simulink model "SMTorqueControl_PdM"  (R2026a)
settings: Solver=FixedStepDiscrete  StopTime=1  FixedStep=Ts  EnableMultiTasking=on
PreLoadFcn:
  | if exist(fullfile(pwd, 'Ortak_Veri_ve_Parametreler'), 'dir'), addpath(fullfile(pwd, 'Ortak_Veri_ve_Parametreler')); end
  | if exist(fullfile(pwd, '..', 'Ortak_Veri_ve_Parametreler'), 'dir'), addpath(fullfile(pwd, '..', 'Ortak_Veri_ve_Parametreler')); end
  | if exist(fullfile(pwd, 'Mat_Dosyalari'), 'dir'), addpath(fullfile(pwd, 'Mat_Dosyalari')); end
  | SMTorqueControlData;
  | if ~exist('Cdc_PdM','var'), Cdc_PdM = Cdc; end;
  | if ~exist('ESR_PdM','var'), ESR_PdM = 1e-4; end;
  | if ~exist('Rbat_PdM','var'), Rbat_PdM = 1e-3; end;
  | if ~exist('Rs_PdM','var'), Rs_PdM = Rs; end;
  | if ~exist('Lad_PdM','var'), Lad_PdM = Lad; end;
  | if ~exist('Rfd_PdM','var'), Rfd_PdM = Rfd; end;
  | if ~exist('Gate_Fault_Mask','var'), Gate_Fault_Mask = [1;1;1;1;1;1]; end;
  | if ~exist('Stator_Unbalance_Gain','var'), Stator_Unbalance_Gain = [1;1;1]; end;
  | if ~exist('Load_Scale_PdM','var'), Load_Scale_PdM = 1.0; end;
  | if ~exist('Sensor_Offset_Drift_PdM','var'), Sensor_Offset_Drift_PdM = [0;0;0]; end;
InitFcn:
  | if exist(fullfile(pwd, 'Ortak_Veri_ve_Parametreler'), 'dir'), addpath(fullfile(pwd, 'Ortak_Veri_ve_Parametreler')); end
  | if exist(fullfile(pwd, '..', 'Ortak_Veri_ve_Parametreler'), 'dir'), addpath(fullfile(pwd, '..', 'Ortak_Veri_ve_Parametreler')); end
  | if exist(fullfile(pwd, 'Mat_Dosyalari'), 'dir'), addpath(fullfile(pwd, 'Mat_Dosyalari')); end
  | SMTorqueControlData;
  | if ~exist('Cdc_PdM','var'), Cdc_PdM = Cdc; end;
  | if ~exist('ESR_PdM','var'), ESR_PdM = 1e-4; end;
  | if ~exist('Rbat_PdM','var'), Rbat_PdM = 1e-3; end;
  | if ~exist('Rs_PdM','var'), Rs_PdM = Rs; end;
  | if ~exist('Lad_PdM','var'), Lad_PdM = Lad; end;
  | if ~exist('Rfd_PdM','var'), Rfd_PdM = Rfd; end;
  | if ~exist('Gate_Fault_Mask','var'), Gate_Fault_Mask = [1;1;1;1;1;1]; end;
  | if ~exist('Stator_Unbalance_Gain','var'), Stator_Unbalance_Gain = [1;1;1]; end;
  | if ~exist('Load_Scale_PdM','var'), Load_Scale_PdM = 1.0; end;
  | if ~exist('Sensor_Offset_Drift_PdM','var'), Sensor_Offset_Drift_PdM = [0;0;0]; end;
undefined symbols (not defined in the file): denZC_id, denZC_if, denZC_iq, ee_sli_rtmsupport, fsw, gcbh, Ibase, ID_MAP, IF_MAP, Ifbase, IQ_MAP, Kaw_id, Kaw_if, Kaw_iq, Ki_id, Ki_if, Ki_iq, Kp_id, Kp_if, Kp_iq, L_base, Lad, Ld, Lq, numZC_id, numZC_if, numZC_iq, p, Pmax, RPM_VECT, Tbase, TQ_VECT, Ts, Tsi, VDC_VECT, Vnom
libraries: nesl_utility x16, fl_lib x11, ee_lib x6, eeGeneralControl x3, eeTransforms x2, deeplib x2, sl_discontinuities x2, SignalEditorBlockLib x2, eeDqVoltageLimiter x1, simulink x1, sl_signal_attributes x1, eePwmGenerator x1
(part 1 of 2)
Description:
  | SM Torque Control
settings Model: Creator=The MathWorks, Inc.  LastModifiedBy=Dogukan.kilinc
settings DataIOCC: MaxDataPoints=210000  SignalLoggingName=logsout_SMTorqueControl
settings SimscapeCC: SimscapeNominalValues="[{\"value\":\"1\",\"unit\":\"A\"},{\"value\":\"1\",\"unit\":\"bar\"},{\"value\":\"1\",\"unit\":\"cm^2\"},{\"value\":\"1\",\"unit\":\"cm^3/s\"},{\"value\":\"1\",\"unit\":\"kJ/kg\"},{\"value\":\"1\",\"unit\":\"kW\"},{\"value\":\"1\",\"unit\":\"l\"},{\"value\":\"1\",\"unit\":\"N\"},{\"value\":\"1\",\"unit\":\"N*m\"},{\"value\":\"1\",\"unit\":\"V\"}]"  SimscapeLogType=none  SimscapeLogSimulationStatistics=on  SimscapeLogName=simlog_SMTorqueControl  SimscapeLogDataHistory=210000.0

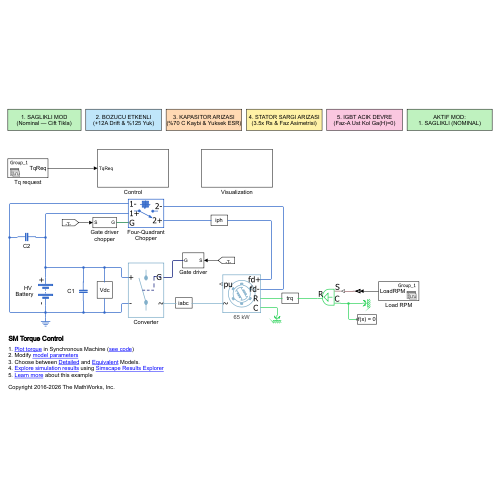
[thumbnail: Simulink's stored preview of the top-level diagram]
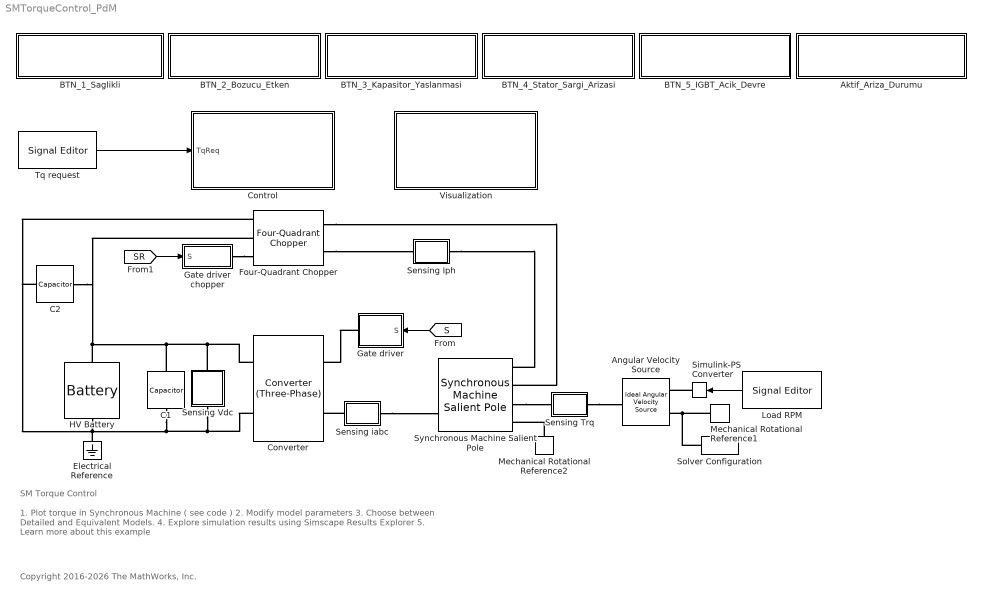
== system SMTorqueControl_PdM ==
  note: SM Torque Control
  note: 1. Plot torque in Synchronous Machine ( see code )
      | 2. Modify model parameters
      | 3. Choose between Detailed and Equivalent Models.
      | 4. Explore simulation results using Simscape Results Explorer
      | 5. Learn more about this example
  note: Copyright 2016-2026 The MathWorks, Inc.
  Aktif_Ariza_Durumu : Subsystem
      settings: OpenFcn=fprintf('[SMTorqueControl_PdM] Soldaki 5 renkli butondan birine cift tiklayarak ariza modunu degistirebilirsiniz.\\n');
      mask Display: disp(['AKTIF MOD:' newline '1. SAGLIKLI (NOMINAL)'])
  Angular Velocity Source : fl_lib/Mechanical/Mechanical Sources/Ideal Angular Velocity Source
  BTN_1_Saglikli : Subsystem
      settings: OpenFcn=|
      | evalin('base', 'if ~exist(''Cdc'',''var''), SMTorqueControlData; end;');
      | evalin('base', 'Cdc_PdM=Cdc; ESR_PdM=1e-3; Rbat_PdM=1e-3; Rs_PdM=Rs; Lad_PdM=Lad; Rfd_PdM=Rfd; Gate_Fault_Mask=[1;1;1;1;1;1]; Stator_Unbalance_Gain=[1;1;1]; Sensor_Offset_Drift_PdM=[0;0;0]; Load_Scale_PdM=1.0;');
      | set_param('SMTorqueControl_PdM/Gate driver/IGBT_Kanal_Maskesi', 'Value', '[1;1;1;1;1;1]');
      | set_param('SMTorqueControl_PdM/Control/Measurements/Stator_Faz_Asimetri_Enjektoru', 'Gain', '[1;1;1]');
      | set_param('SMTorqueControl_PdM/Control/Measurements/Sensor_Bozucu_Ofset', 'Value', '[0;0;0]');
      | set_param('SMTorqueControl_PdM/Control/Yuk_Olcekleyici', 'Gain', '1.0');
      | set_param('SMTorqueControl_PdM/Aktif_Ariza_Durumu', 'MaskDisplay', 'disp([''AKTIF MOD:'' newline ''1. SAGLIKLI (NOMINAL)''])', 'BackgroundColor', '[0.75 0.95 0.75]');
      | if strcmp(get_param('SMTorqueControl_PdM','SimulationStatus'),'running'), set_param('SMTorqueControl_PdM','SimulationCommand','update'); end;
      | fprintf('[SMTorqueControl_PdM] >>> Mod 1 Secildi: SAGLIKLI (NOMINAL) MOD aktif!\n');
      mask Display: disp('1. SAGLIKLI MOD\n(Nominal — Cift Tikla)')
  BTN_2_Bozucu_Etken : Subsystem
      settings: OpenFcn=|
      | evalin('base', 'if ~exist(''Cdc'',''var''), SMTorqueControlData; end;');
      | evalin('base', 'Cdc_PdM=Cdc; ESR_PdM=1e-3; Rbat_PdM=1e-3; Rs_PdM=Rs; Lad_PdM=Lad; Rfd_PdM=Rfd; Gate_Fault_Mask=[1;1;1;1;1;1]; Stator_Unbalance_Gain=[1.04;0.98;0.98]; Sensor_Offset_Drift_PdM=[12;-6;-6]; Load_Scale_PdM=1.25;');
      | set_param('SMTorqueControl_PdM/Gate driver/IGBT_Kanal_Maskesi', 'Value', '[1;1;1;1;1;1]');
      | set_param('SMTorqueControl_PdM/Control/Measurements/Stator_Faz_Asimetri_Enjektoru', 'Gain', '[1.04;0.98;0.98]');
      | set_param('SMTorqueControl_PdM/Control/Measurements/Sensor_Bozucu_Ofset', 'Value', '[12;-6;-6]');
      | set_param('SMTorqueControl_PdM/Control/Yuk_Olcekleyici', 'Gain', '1.25');
      | set_param('SMTorqueControl_PdM/Aktif_Ariza_Durumu', 'MaskDisplay', 'disp([''AKTIF MOD:'' newline ''2. BOZUCU ETKEN (+12A, %125)''])', 'BackgroundColor', '[0.75 0.90 0.98]');
      | if strcmp(get_param('SMTorqueControl_PdM','SimulationStatus'),'running'), set_param('SMTorqueControl_PdM','SimulationCommand','update'); end;
      | fprintf('[SMTorqueControl_PdM] >>> Mod 2 Secildi: BOZUCU ETKENLI SAGLIKLI MOD (+12A Drift, %%125 Yuk) aktif!\n');
      mask Display: disp('2. BOZUCU ETKENLI\n(+12A Drift & %125 Yuk)')
  BTN_3_Kapasitor_Yaslanmasi : Subsystem
      settings: OpenFcn=|
      | evalin('base', 'if ~exist(''Cdc'',''var''), SMTorqueControlData; end;');
      | evalin('base', 'Cdc_PdM=0.30*Cdc; ESR_PdM=0.08; Rbat_PdM=0.18; Rs_PdM=Rs; Lad_PdM=Lad; Rfd_PdM=Rfd; Gate_Fault_Mask=[1;1;1;1;1;1]; Stator_Unbalance_Gain=[1;1;1]; Sensor_Offset_Drift_PdM=[0;0;0]; Load_Scale_PdM=1.0;');
      | set_param('SMTorqueControl_PdM/Gate driver/IGBT_Kanal_Maskesi', 'Value', '[1;1;1;1;1;1]');
      | set_param('SMTorqueControl_PdM/Control/Measurements/Stator_Faz_Asimetri_Enjektoru', 'Gain', '[1;1;1]');
      | set_param('SMTorqueControl_PdM/Control/Measurements/Sensor_Bozucu_Ofset', 'Value', '[0;0;0]');
      | set_param('SMTorqueControl_PdM/Control/Yuk_Olcekleyici', 'Gain', '1.0');
      | set_param('SMTorqueControl_PdM/Aktif_Ariza_Durumu', 'MaskDisplay', 'disp([''AKTIF MOD:'' newline ''3. KAPASITOR YASLANMASI''])', 'BackgroundColor', '[1.00 0.85 0.70]');
      | if strcmp(get_param('SMTorqueControl_PdM','SimulationStatus'),'running'), set_param('SMTorqueControl_PdM','SimulationCommand','update'); end;
      | fprintf('[SMTorqueControl_PdM] >>> Mod 3 Secildi: DC-LINK KAPASITOR YASLANMASI aktif!\n');
      mask Display: disp('3. KAPASITOR ARIZASI\n(%70 C Kaybi & Yuksek ESR)')
  BTN_4_Stator_Sargi_Arizasi : Subsystem
      settings: OpenFcn=|
      | evalin('base', 'if ~exist(''Cdc'',''var''), SMTorqueControlData; end;');
      | evalin('base', 'Cdc_PdM=Cdc; ESR_PdM=1e-3; Rbat_PdM=1e-3; Rs_PdM=3.5*Rs; Lad_PdM=0.82*Lad; Rfd_PdM=1.4*Rfd; Gate_Fault_Mask=[1;1;1;1;1;1]; Stator_Unbalance_Gain=[1.12;0.94;0.94]; Sensor_Offset_Drift_PdM=[0;0;0]; Load_Scale_PdM=1.0;');
      | set_param('SMTorqueControl_PdM/Gate driver/IGBT_Kanal_Maskesi', 'Value', '[1;1;1;1;1;1]');
      | set_param('SMTorqueControl_PdM/Control/Measurements/Stator_Faz_Asimetri_Enjektoru', 'Gain', '[1.12;0.94;0.94]');
      | set_param('SMTorqueControl_PdM/Control/Measurements/Sensor_Bozucu_Ofset', 'Value', '[0;0;0]');
      | set_param('SMTorqueControl_PdM/Control/Yuk_Olcekleyici', 'Gain', '1.0');
      | set_param('SMTorqueControl_PdM/Aktif_Ariza_Durumu', 'MaskDisplay', 'disp([''AKTIF MOD:'' newline ''4. STATOR SARGI ARIZASI''])', 'BackgroundColor', '[1.00 0.95 0.65]');
      | if strcmp(get_param('SMTorqueControl_PdM','SimulationStatus'),'running'), set_param('SMTorqueControl_PdM','SimulationCommand','update'); end;
      | fprintf('[SMTorqueControl_PdM] >>> Mod 4 Secildi: STATOR SARGI ARIZASI & FAZ ASIMETRISI aktif!\n');
      mask Display: disp('4. STATOR SARGI ARIZASI\n(3.5x Rs & Faz Asimetrisi)')
  BTN_5_IGBT_Acik_Devre : Subsystem
      settings: OpenFcn=|
      | evalin('base', 'if ~exist(''Cdc'',''var''), SMTorqueControlData; end;');
      | evalin('base', 'Cdc_PdM=Cdc; ESR_PdM=1e-3; Rbat_PdM=1e-3; Rs_PdM=Rs; Lad_PdM=Lad; Rfd_PdM=Rfd; Gate_Fault_Mask=[0;1;1;1;1;1]; Stator_Unbalance_Gain=[1;1;1]; Sensor_Offset_Drift_PdM=[0;0;0]; Load_Scale_PdM=1.0;');
      | set_param('SMTorqueControl_PdM/Gate driver/IGBT_Kanal_Maskesi', 'Value', '[0;1;1;1;1;1]');
      | set_param('SMTorqueControl_PdM/Control/Measurements/Stator_Faz_Asimetri_Enjektoru', 'Gain', '[1;1;1]');
      | set_param('SMTorqueControl_PdM/Control/Measurements/Sensor_Bozucu_Ofset', 'Value', '[0;0;0]');
      | set_param('SMTorqueControl_PdM/Control/Yuk_Olcekleyici', 'Gain', '1.0');
      | set_param('SMTorqueControl_PdM/Aktif_Ariza_Durumu', 'MaskDisplay', 'disp([''AKTIF MOD:'' newline ''5. INVERTER IGBT ARIZASI''])', 'BackgroundColor', '[0.98 0.78 0.88]');
      | if strcmp(get_param('SMTorqueControl_PdM','SimulationStatus'),'running'), set_param('SMTorqueControl_PdM','SimulationCommand','update'); end;
      | fprintf('[SMTorqueControl_PdM] >>> Mod 5 Secildi: INVERTER A-FAZI UST IGBT ACIK DEVRE ARIZASI aktif!\n');
      mask Display: disp('5. IGBT ACIK DEVRE\n(Faz-A Ust Kol Ga(H)=0)')
  C1 : fl_lib/Electrical/Electrical Elements/Capacitor  c=Cdc_PdM F  r=ESR_PdM Ohm  g=0 1/Ohm  i_specify=off  i_priority=None  i=0 A  i_nominal_specify=off  i_nominal_value=1  i_nominal_unit=A  v_specify=off  v_priority=None  v=0 V  v_nominal_specify=off  v_nominal_value=1  v_nominal_unit=V  vc_specify=on  vc_priority=None  vc=Vnom V  vc_nominal_specify=off  vc_nominal_value=1  vc_nominal_unit=V
  C2 : fl_lib/Electrical/Electrical Elements/Capacitor  c=Cdc_PdM F  r=ESR_PdM Ohm  g=0 1/Ohm  i_specify=off  i_priority=None  i=0 A  i_nominal_specify=off  i_nominal_value=1  i_nominal_unit=A  v_specify=off  v_priority=None  v=0 V  v_nominal_specify=off  v_nominal_value=1  v_nominal_unit=V  vc_specify=on  vc_priority=None  vc=Vnom V  vc_nominal_specify=off  vc_nominal_value=1  vc_nominal_unit=V
  Control : Subsystem
  Converter : ee_lib/Semiconductors & Converters/Converters/Converter (Three-Phase)  port_option=ee.enum.threePhasePort.composite  fidelity_option=ee.enum.converters.fidelity.detailed  device_type=2  showThermalPort=false  K=0  Vth=0.5 V  Vgt=1 V  Vgt_off=-1 V  Ih=1 A  Vf=0.8 V  Ron=0.001 Ohm  Rds=0.001 Ohm  Goff=1e-5 1/Ohm  Eon_scalar=22.86e-3 J  Eoff_scalar=17.14e-3 J  Eoff_natural_commutation=10e-3 J  Voff=300 V  Iout_scalar=600 A  onCurrentMeasDelay=0 s  useCurrentFromPreviousCycle=false  useVoltageFromPreviousCycle=false  diode_param=2  diode_Vf=0.8 V  diode_Ron=0.001 Ohm  diode_Goff=1e-5 1/Ohm  diode_C=50 nF  diode_iRM=-235 A  diode_iF=300 A  diode_idot=-50 A/us  diode_trr_param=1  diode_trr_factor=3  diode_trr=15 us  diode_Qrr=1.5e+3 s*uA  diode_rec_loss_model=ee.enum.diode.reverseRecoveryModel.fixed  diode_ErecVal=0 J  diode_scaleWithIandV=false  diode_ErecMat=zeros(2, 3) J  diode_TjrecVec=[298.15, 398.15] K  diode_IfrecVec=[.1, 1, 10] A  diode_IrecVal=10 A  diode_VrecVal=10 V  diode_tFilter=1 / 1000 / 100 s  thermal_network_parameterization=ee.enum.thermalNetworkTopology.external  Rth=[.08, .5] K/W  Rth_Cauer=[.08, .1, .5] K/W  Rth_Foster=[.08, .14, .22, .16] K/W  thermal_mass_parameterization=ee.enum.thermalNetwork.timeconstant  thermal_mass=[.01, .5] J/K  thermal_mass_Cauer=[.01, .1, .5] J/K  thermal_mass_Foster=[.001, .005, .05, .5] J/K  thermal_time_constant=[.001, .2] s  thermal_time_constant_Cauer=[.001, .1, .2] s  thermal_time_constant_Foster=[7e-05, .0007, .01, .08] s  thermal_mass_initial_temperatures=[25, 25] degC  thermal_mass_initial_temperatures_Cauer=[25, 25, 25] degC  junction_thermal_mass=0.01 J/K  Tvec_initial_Foster=[25, 25, 25, 25] degC  snubber_type=0  Cs=1e-7 F  Rs=0.1 Ohm  Vce_loss=[0, 150, 300] V
  Electrical Reference : fl_lib/Electrical/Electrical Elements/Electrical Reference
  Four-Quadrant Chopper : ee_lib/Semiconductors & Converters/Converters/Four-Quadrant Chopper  fidelity_option=ee.enum.converters.fidelity.detailed  device_type=3  showThermalPort=false  Vgt=1 V  Vgt_off=-1 V  Ih=1 A  Vf=0.8 V  Ron=0.001 Ohm  Rds=0.001 Ohm  Goff=1e-5 1/Ohm  Vth=0.5 V  K=0  Eon_scalar=22.86e-3 J  Eoff_scalar=17.14e-3 J  Eoff_natural_commutation=10e-3 J  Voff=300 V  Iout_scalar=600 A  onCurrentMeasDelay=0 s  useCurrentFromPreviousCycle=false  useVoltageFromPreviousCycle=false  diode_param=2  diode_Vf=0.8 V  diode_Ron=0.001 Ohm  diode_Goff=1e-5 1/Ohm  diode_C=50 nF  diode_iRM=-235 A  diode_iF=300 A  diode_idot=-50 A/us  diode_trr_param=1  diode_trr_factor=3  diode_trr=15 us  diode_Qrr=1500 s*uA  diode_rec_loss_model=ee.enum.diode.reverseRecoveryModel.fixed  diode_ErecVal=0 J  diode_scaleWithIandV=false  diode_ErecMat=zeros(2, 3) J  diode_TjrecVec=[298.15, 398.15] K  diode_IfrecVec=[.1, 1, 10] A  diode_IrecVal=10 A  diode_VrecVal=10 V  diode_tFilter=1 / 1000 / 100 s  thermal_network_parameterization=ee.enum.thermalNetworkTopology.external  Rth=[.08, .5] K/W  Rth_Cauer=[.08, .1, .5] K/W  Rth_Foster=[.08, .14, .22, .16] K/W  thermal_mass_parameterization=ee.enum.thermalNetwork.timeconstant  thermal_mass=[.01, .5] J/K  thermal_mass_Cauer=[.01, .1, .5] J/K  thermal_mass_Foster=[.001, .005, .05, .5] J/K  thermal_time_constant=[.001, .2] s  thermal_time_constant_Cauer=[.001, .1, .2] s  thermal_time_constant_Foster=[7e-05, .0007, .01, .08] s  thermal_mass_initial_temperatures=[25, 25] degC  thermal_mass_initial_temperatures_Cauer=[25, 25, 25] degC  junction_thermal_mass=0.01 J/K  Tvec_initial_Foster=[25, 25, 25, 25] degC  snubber_type=0  Cs=1e-7 F  Rs=0.1 Ohm
  Gate driver : Subsystem
  Gate driver chopper : Subsystem
  HV Battery : batteryecm_lib/Battery  Vnom=Vnom V  prm_dir=1  R1_dis=2 Ohm  R1_ch=2 Ohm  R1=Rbat_PdM Ohm  prm_AH=1  AH=300 hr*A  V1=330 V  AH1=100 hr*A  prm_R2=1  R2=2000 Ohm  Tmeas=298.15 K  charge_measurement_port=simscape.enum.battery.enable.no  prm_dyn=1  Rp1=0.005 Ohm  tau1=30 s  Rp2=0.005 Ohm  tau2=30 s  Rp3=0.005 Ohm  tau3=30 s  Rp4=0.005 Ohm  tau4=30 s  Rp5=0.005 Ohm  tau5=30 s  prm_fade=1  N_fade=100  AH_fade=45 hr*A  R1_fade=2.02 Ohm  R1_ch_fade=2.02 Ohm  V1_fade=10.35 V  prm_age=1  prm_age_OCV=1  OCV_age=0.9  SOC_age=60  Tmeas_age=298.15 K  delta_time_age_vec=[0] d  temperature_age_vec=[273] K  OCV_scaling_age=2.2134e6  OCV_offset_age=1.632e6  temp_exp_age=0.515833569 V  t_exp_age=0.75  Vnom_T2=12 V  R1_T2=2.2 Ohm  R1_T2_dis=2.2 Ohm  R1_T2_ch=2.2 Ohm  V1_T2=11.4 V  R2_T2=2200 Ohm  Rp1_T2=0.005 Ohm  tau1_T2=30 s  Rp2_T2=0.005 Ohm  tau2_T2=30 s  Rp3_T2=0.005 Ohm  tau3_T2=30 s  Rp4_T2=0.005 Ohm  tau4_T2=30 s  Rp5_T2=0.005 Ohm  tau5_T2=30 s  Tmeas2=273.15 K  thermal_port=simscape.enum.thermaleffects.omit  thermal_mass=30000 J/K  i_specify=off  i_priority=None  i=0 A  i_nominal_specify=off  i_nominal_value=1  i_nominal_unit=A  v_specify=off  v_priority=None  v=0 V  v_nominal_specify=off  v_nominal_value=1  v_nominal_unit=V  charge_specify=on  charge_priority=High  charge=AH0 hr*A  charge_nominal_specify=off  charge_nominal_value=1  charge_nominal_unit=A*hr  num_cycles_specify=off  num_cycles_priority=High  num_cycles=0  num_cycles_nominal_specify=off  num_cycles_nominal_value=1  num_cycles_nominal_unit=1  temperature_specify=off  temperature_priority=High  temperature=298.15 K  temperature_nominal_specify=off  temperature_nominal_value=1  temperature_nominal_unit=K
  Load RPM : SignalEditorBlockLib/Signal Editor  FileName=SMTorqueControlLoadRPM.mat  ActiveScenario=Group_1  ActiveSignal=LoadRPM  IsBus=off  OutputBusObjectStr=Bus: BusObject  SampleTime=0  OutputAfterFinalValue=Extrapolation  Unit=inherit  PreserveSignalName=on  ApplySigPropsToAllScenarios=on  ApplySigPropsToAllSignals=off  SignalPropertySource=Dialog parameters
  Mechanical Rotational Reference1 : fl_lib/Mechanical/Rotational Elements/Mechanical Rotational Reference
  Mechanical Rotational Reference2 : fl_lib/Mechanical/Rotational Elements/Mechanical Rotational Reference
  Sensing Iph : Subsystem
      mask Display: disp('iph')
  Sensing Trq : Subsystem
      mask Display: disp('trq')
  Sensing Vdc : Subsystem
      mask Display: disp('Vdc')
  Sensing iabc : Subsystem
      mask Display: disp('iabc')
  Simulink-PS Converter : nesl_utility/Simulink-PS Converter  PhysicalDomain=network_engine_domain  SubClassName=ps_input  LeftPortType=input  RightPortType=output  PseudoPeriodic=off  Frequencies=[]  NoiseDistribution=none  NoiseParameters=[]  Unit=rpm  AffineConversion=off  FilteringAndDerivatives=zero  SimscapeFilterOrder=1  InputFilterTimeConstant=0.001  UdotUserProvided=1
  Solver Configuration : nesl_utility/Solver Configuration  PhysicalDomain=network_engine_domain  SubClassName=solver  LeftPortType=input  RightPortType=generic  Tones=[]  Harmonics=[]  SimulateNoise=off  Profile=off  UseLocalSampling=off  EnableSwitchedLinearOptims=on  FrequencyDomain=off  UseCCode=off  RelTol=0.001  AbsTol=1e-06  MinStep=1e-09  ToWorkspace=off  RevertToSquareIcSolve=off  NumHomotopyIterations=100  PhasorMode=off  PhasorModeNumHarmonics=1  ConsistencySolver=NEWTON_FTOL  CanonicalOrdering=UNORDERED  OptimizeIntermediates=UNOPTIMIZED  IndexReductionMethod=DerivativeReplacement  DoDC=off  ResidualTolerance=1e-9  ConsistencyTolSource=GLOBAL  ConsistencyAbsTol=0.001  ConsistencyRelTol=0.001  ConsistencyTolFactor=0.001  UseLocalSolver=on  LocalSolverChoice=NE_BACKWARD_EULER_ADVANCER  ResolveIndetEquations=on  FunctionEvalNumThread=1  LocalSolverSampleTime=Ts  DoFixedCost=on  MaxNonlinIter=4  MaxModeIter=2  ComputeImpulses=off  ImpulseIterations=2  LinearAlgebra=auto  LinearAlgebraNumThread=0  EquationFormulation=NE_TIME_EF  DelaysMemoryBudget=1024  AutomaticFiltering=on  FilteringTimeConstant=0.001  PartitionStorageMethod=AS_NEEDED  PartitionMemoryBudget=1024  PartitionMethod=FAST  MultibodyUseLocalSolver=off  MultibodyLocalSolverChoice=ODE1  MultibodyLocalSolverSampleTime=0.001
  Synchronous Machine Salient Pole : ee_lib/Electromechanical/Synchronous/Synchronous Machine Salient Pole  port_option=ee.enum.threePhasePort.composite  SRated=Pmax W  VRated=Vr V  FRated=fr Hz  nPolePairs=p  param_option=ee.enum.sm.parameterization.fundamental  fieldCircuitParameterization_option=2  baseEfd=272 V  baseIfd=Ifbase A  zero_sequence=ee.enum.park.zerosequence.exclude  axes_param=ee.enum.rotorangle.daxis  Ladu=Lad_PdM  Laqu=Laq  L0=L0  Ll=Ll  Ra=Rs_PdM  Lfd=Lfd  Rfd=Rfd_PdM  L1d=0.1  R1d=0.254  L1q=0.1567  R1q=0.328  Xl=0.15  Xd=1.05  Xq=0.7  X0=0.15  Xdd=0.35  Xddd=0.25  Xqdd=0.325  d_option=ee.enum.circuit.open  Td0d=5.25 s  Tdd=1.75 s  Td0dd=0.03 s  Tddd=0.0214 s  q_option=ee.enum.circuit.open  Tq0dd=0.05 s  Tqdd=0.0232 s  saturation_option=0  saturation_ifd=[0.0, 0.48, 0.76, 1.38, 1.79]  saturation_Vag=[0.0, 0.43, 0.59, 0.71, 0.76]  initialization_option=1  source_type=ee.enum.sm.load_flow_source_type.Swing  Vmag0=Vr V  Vang0=0 deg  Pt0=0 V*A  Qt0=0 V*A  minimum_pu=0.95  phase_search_range=[-30, 30] deg  gmin=1e-6 S  connection_option=ee.enum.Connection.wye  num_q_dampers=1  rotor_offset=-pi / 2 rad  pu_psid_specify=on  pu_psid_priority=High  pu_psid=0  pu_psid_nominal_specify=off  pu_psid_nominal_value=1  pu_psid_nominal_unit=1  pu_psiq_specify=on  pu_psiq_priority=High  pu_psiq=0  pu_psiq_nominal_specify=off  pu_psiq_nominal_value=1  pu_psiq_nominal_unit=1  pu_psifd_specify=on  pu_psifd_priority=High  pu_psifd=0  pu_psifd_nominal_specify=off  pu_psifd_nominal_value=1  pu_psifd_nominal_unit=1  pu_psi1d_specify=on  pu_psi1d_priority=High  pu_psi1d=0  pu_psi1d_nominal_specify=off  pu_psi1d_nominal_value=1  pu_psi1d_nominal_unit=1  pu_psi1q_specify=on  pu_psi1q_priority=High  pu_psi1q=0  pu_psi1q_nominal_specify=off  pu_psi1q_nominal_value=1  pu_psi1q_nominal_unit=1  angular_position_diff_specify=on  angular_position_diff_priority=High  angular_position_diff=-pi/2/p rad  angular_position_diff_nominal_specify=off  angular_position_diff_nominal_value=1  angular_position_diff_nominal_unit=deg  Tmeas=298.15 K  alpha=3.93e-3 1/K  stator_thermal_mass=100 J/K  rotor_thermal_mass=200 J/K  temperatureA_specify=off  temperatureA_priority=High  temperatureA=25 degC  temperatureA_nominal_specify=off  temperatureA_nominal_value=1  temperatureA_nominal_unit=degC  temperatureB_specify=off  temperatureB_priority=High  temperatureB=25 degC  temperatureB_nominal_specify=off  temperatureB_nominal_value=1  temperatureB_nominal_unit=degC  temperatureC_specify=off  temperatureC_priority=High  temperatureC=25 degC  temperatureC_nominal_specify=off  temperatureC_nominal_value=1  temperatureC_nominal_unit=degC  temperatureR_specify=off  temperatureR_priority=High  temperatureR=25 degC  temperatureR_nominal_specify=off  temperatureR_nominal_value=1  temperatureR_nominal_unit=degC
      settings: AttributesFormatString=65 kW
  Tq request : SignalEditorBlockLib/Signal Editor  FileName=SMTorqueControlTorqueRequest.mat  ActiveScenario=Group_1  ActiveSignal=TqReq  IsBus=off  OutputBusObjectStr=Bus: BusObject  SampleTime=0  OutputAfterFinalValue=Extrapolation  Unit=inherit  PreserveSignalName=on  ApplySigPropsToAllScenarios=on  ApplySigPropsToAllSignals=off  SignalPropertySource=Dialog parameters
  Visualization : Subsystem
  wires:
  [S] -> Gate driver/1(S)
  Load RPM/1 -> Simulink-PS Converter/1
  [SR] -> Gate driver chopper/1(S)
  Tq request/1 -> Control/1(TqReq)
  connections:
  Sensing Trq/RConn1 -- Angular Velocity Source/LConn1
  Converter/RConn2 -- Sensing Vdc/RConn1 -- Four-Quadrant Chopper/LConn3 -- C2/RConn1 -- HV Battery/RConn1 -- Electrical Reference/LConn1 -- C1/RConn1
  Converter/RConn1 -- Sensing Vdc/LConn1 -- Four-Quadrant Chopper/LConn2 -- C2/LConn1 -- HV Battery/LConn1 -- C1/LConn1
  Gate driver/RConn1 -- Converter/LConn1
  Simulink-PS Converter/RConn1 -- Angular Velocity Source/RConn1
  Synchronous Machine Salient Pole/LConn3 -- Sensing Trq/LConn1
  Mechanical Rotational Reference1/LConn1 -- Solver Configuration/RConn1 -- Angular Velocity Source/RConn2
  Four-Quadrant Chopper/RConn1 -- Sensing Iph/LConn1
  Four-Quadrant Chopper/RConn2 -- Synchronous Machine Salient Pole/LConn2
  Sensing Iph/RConn1 -- Synchronous Machine Salient Pole/LConn1
  Sensing iabc/LConn1 -- Converter/LConn2
  Sensing iabc/RConn1 -- Synchronous Machine Salient Pole/RConn2
  Gate driver chopper/RConn1 -- Four-Quadrant Chopper/LConn1
  Mechanical Rotational Reference2/LConn1 -- Synchronous Machine Salient Pole/LConn4

== system SMTorqueControl_PdM/Aktif_Ariza_Durumu ==

== system SMTorqueControl_PdM/BTN_1_Saglikli ==

== system SMTorqueControl_PdM/BTN_2_Bozucu_Etken ==

== system SMTorqueControl_PdM/BTN_3_Kapasitor_Yaslanmasi ==

== system SMTorqueControl_PdM/BTN_4_Stator_Sargi_Arizasi ==

== system SMTorqueControl_PdM/BTN_5_IGBT_Acik_Devre ==

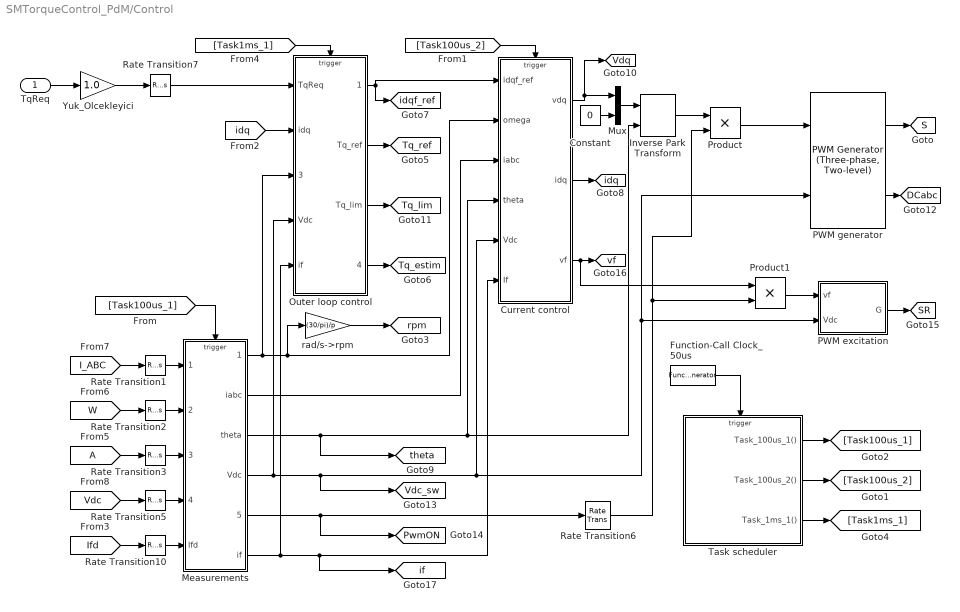
== system SMTorqueControl_PdM/Control ==
  TqReq : Inport
  Constant : Constant  Value=0  SampleTime=-1
  Current control : Subsystem
  From5 : From  TagVisibility=global
  Function-Call Clock_50us : FunctionCallGenerator  SampleTime=5e-5
  Inverse Park Transform : eeTransforms/Inverse Park Transform  AxisAlignment=Q-axis  PowerInvariant=off
  Measurements : Subsystem
  Mux : Mux  Inputs=2
  Outer loop control : Subsystem
  PWM excitation : Subsystem
  PWM generator : eePwmGeneratorTwoLevel/PWM Generator (Three-phase, Two-level)  PWMMode=Continuous PWM (CPWM)  CPWMMode=SVM: space vector modulation  DPWMMode=60 DPWM: 60 degree discontinuous PWM  fsw=fsw  Ts=Ts
  Product : Product
  Product1 : Product
  Rate Transition{1..3,5..7,10} (7 alike) : RateTransition
  Task scheduler : Stateflow chart  TreatAsAtomicUnit=on
  Yuk_Olcekleyici : Gain  Gain=1.0
  rad/s->rpm : Gain  Gain=(30/pi)/p
  tag scope: DCabc=global, PwmON=global, S=global, SR=global, Tq_estim=global, Tq_lim=global, Tq_ref=global, Vdc_sw=global, Vdq=global, idq=global, idqf_ref=global, if=global, rpm=global, theta=global, vf=global
  wires:
  [Ifd] -> Rate Transition10/1
  [W] -> Rate Transition2/1
  [idq] -> Outer loop control/2(idq)
  [Task100us_1] -> Measurements/Trigger
  Measurements/5(PwmON) -> Rate Transition6/1, [PwmON]
  Rate Transition1/1 -> Measurements/1(iabc_m)
  PWM generator/2 -> [DCabc]
  [I_ABC] -> Rate Transition1/1
  Rate Transition6/1 -> Product1/2, Product/2
  [Task100us_2] -> Current control/Trigger
  Measurements/2(iabc) -> Current control/3(iabc)
  Outer loop control/4(Tq_estim) -> [Tq_estim]
  Current control/3(vf) -> Product1/1, [vf]
  Measurements/1(omega) -> rad/s->rpm/1, Current control/2(omega), Outer loop control/3(omega)
  rad/s->rpm/1 -> [rpm]
  Current control/2(idq) -> [idq]
  Rate Transition10/1 -> Measurements/5(Ifd)
  Task scheduler/2(Task_100us_2()) -> [Task100us_2]
  From5/1 -> Rate Transition3/1
  Measurements/3(theta) -> [theta], Inverse Park Transform/2, Current control/4(theta)
  Outer loop control/2(Tq_ref) -> [Tq_ref]
  Task scheduler/1(Task_100us_1()) -> [Task100us_1]
  [Task1ms_1] -> Outer loop control/Trigger
  Rate Transition2/1 -> Measurements/2(omega_m)
  Task scheduler/3(Task_1ms_1()) -> [Task1ms_1]
  Measurements/4(Vdc) -> [Vdc_sw], PWM generator/2, PWM excitation/2(Vdc), Current control/5(Vdc), Outer loop control/4(Vdc)
  [Vdc] -> Rate Transition5/1
  Rate Transition5/1 -> Measurements/4(Vdc_m)
  PWM generator/1 -> [S]
  Rate Transition3/1 -> Measurements/3(theta_m)
  Outer loop control/3(Tq_lim) -> [Tq_lim]
  Measurements/6(if) -> [if], Current control/6(If), Outer loop control/5(if)
  PWM excitation/1(G) -> [SR]
  Function-Call Clock_50us/1 -> Task scheduler/Trigger
  Outer loop control/1(idqf_ref) -> Current control/1(idqf_ref), [idqf_ref]
  Constant/1 -> Mux/2
  Mux/1 -> Inverse Park Transform/1
  Current control/1(vdq) -> [Vdq], Mux/1
  Product/1 -> PWM generator/1
  Inverse Park Transform/1 -> Product/1
  Product1/1 -> PWM excitation/1(vf)
  TqReq/1 -> Yuk_Olcekleyici/1
  Yuk_Olcekleyici/1 -> Rate Transition7/1
  Rate Transition7/1 -> Outer loop control/1(TqReq)

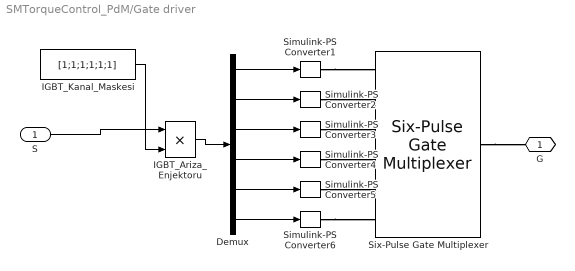
== system SMTorqueControl_PdM/Gate driver ==
  S : Inport
  Demux : Demux  Outputs=6
  IGBT_Ariza_Enjektoru : Product  Inputs=**
  IGBT_Kanal_Maskesi : Constant  Value=[1;1;1;1;1;1]
  Simulink-PS Converter{1..6} (6 alike) : nesl_utility/Simulink-PS Converter  PhysicalDomain=network_engine_domain  SubClassName=ps_input  LeftPortType=input  RightPortType=output  PseudoPeriodic=off  Frequencies=[]  NoiseDistribution=none  NoiseParameters=[]  Unit=1  AffineConversion=off  FilteringAndDerivatives=zero  SimscapeFilterOrder=1  InputFilterTimeConstant=0.001  UdotUserProvided=1
  Six-Pulse Gate Multiplexer : ee_lib/Semiconductors & Converters/Converters/Six-Pulse Gate Multiplexer  port_option=ee.enum.controlport.ps
  G : PMIOPort  Side=Right
  wires:
  Demux/1 -> Simulink-PS Converter1/1
  Demux/4 -> Simulink-PS Converter4/1
  Demux/2 -> Simulink-PS Converter2/1
  Demux/3 -> Simulink-PS Converter3/1
  Demux/5 -> Simulink-PS Converter5/1
  Demux/6 -> Simulink-PS Converter6/1
  S/1 -> IGBT_Ariza_Enjektoru/1
  IGBT_Kanal_Maskesi/1 -> IGBT_Ariza_Enjektoru/2
  IGBT_Ariza_Enjektoru/1 -> Demux/1
  connections:
  Six-Pulse Gate Multiplexer/RConn1 -- G/RConn1
  Simulink-PS Converter1/RConn1 -- Six-Pulse Gate Multiplexer/LConn1
  Simulink-PS Converter3/RConn1 -- Six-Pulse Gate Multiplexer/LConn3
  Simulink-PS Converter5/RConn1 -- Six-Pulse Gate Multiplexer/LConn5
  Simulink-PS Converter6/RConn1 -- Six-Pulse Gate Multiplexer/LConn6
  Simulink-PS Converter4/RConn1 -- Six-Pulse Gate Multiplexer/LConn4
  Simulink-PS Converter2/RConn1 -- Six-Pulse Gate Multiplexer/LConn2

== system SMTorqueControl_PdM/Gate driver chopper ==
  S : Inport
  Demux : Demux  Outputs=2
  Four-Pulse Gate Multiplexer : ee_lib/Semiconductors & Converters/Converters/Four-Pulse Gate Multiplexer  port_option=ee.enum.controlport.ps
  Simulink-PS Converter1 : nesl_utility/Simulink-PS Converter  PhysicalDomain=network_engine_domain  SubClassName=ps_input  LeftPortType=input  RightPortType=output  PseudoPeriodic=off  Frequencies=[]  NoiseDistribution=none  NoiseParameters=[]  Unit=1  AffineConversion=off  FilteringAndDerivatives=zero  SimscapeFilterOrder=1  InputFilterTimeConstant=0.001  UdotUserProvided=1
  Simulink-PS Converter2 : nesl_utility/Simulink-PS Converter  PhysicalDomain=network_engine_domain  SubClassName=ps_input  LeftPortType=input  RightPortType=output  PseudoPeriodic=off  Frequencies=[]  NoiseDistribution=none  NoiseParameters=[]  Unit=1  AffineConversion=off  FilteringAndDerivatives=zero  SimscapeFilterOrder=1  InputFilterTimeConstant=0.001  UdotUserProvided=1
  G : PMIOPort  Side=Right
  wires:
  Demux/2 -> Simulink-PS Converter2/1
  S/1 -> Demux/1
  Demux/1 -> Simulink-PS Converter1/1
  connections:
  Simulink-PS Converter2/RConn1 -- Four-Pulse Gate Multiplexer/LConn2 -- Four-Pulse Gate Multiplexer/LConn3
  Four-Pulse Gate Multiplexer/LConn1 -- Four-Pulse Gate Multiplexer/LConn4 -- Simulink-PS Converter1/RConn1
  G/RConn1 -- Four-Pulse Gate Multiplexer/RConn1

== system SMTorqueControl_PdM/Sensing Iph ==
  Current Sensor : fl_lib/Electrical/Electrical Sensors/Current Sensor
  PS-Simulink Converter : nesl_utility/PS-Simulink Converter  PhysicalDomain=network_engine_domain  SubClassName=ps_output  LeftPortType=input  RightPortType=output  PseudoPeriodic=off  Frequencies=[]  VectorFormat=1-D array  Unit=1  AffineConversion=off
  + : PMIOPort  Side=Left
  - : PMIOPort  Port=2  Side=Right
  tag scope: Ifd=global
  wires:
  PS-Simulink Converter/1 -> [Ifd]
  connections:
  Current Sensor/LConn1 -- +/RConn1
  Current Sensor/RConn2 -- -/RConn1
  PS-Simulink Converter/LConn1 -- Current Sensor/RConn1

== system SMTorqueControl_PdM/Sensing Trq ==
  Goto3 : Goto  TagVisibility=global
  Mechanical Rotational Reference2 : fl_lib/Mechanical/Rotational Elements/Mechanical Rotational Reference
  PS-Simulink Converter1 : nesl_utility/PS-Simulink Converter  PhysicalDomain=network_engine_domain  SubClassName=ps_output  LeftPortType=input  RightPortType=output  PseudoPeriodic=off  Frequencies=[]  VectorFormat=1-D array  Unit=rad/s  AffineConversion=off
  PS-Simulink Converter2 : nesl_utility/PS-Simulink Converter  PhysicalDomain=network_engine_domain  SubClassName=ps_output  LeftPortType=input  RightPortType=output  PseudoPeriodic=off  Frequencies=[]  VectorFormat=1-D array  Unit=rad  AffineConversion=off
  PS-Simulink Converter3 : nesl_utility/PS-Simulink Converter  PhysicalDomain=network_engine_domain  SubClassName=ps_output  LeftPortType=input  RightPortType=output  PseudoPeriodic=off  Frequencies=[]  VectorFormat=1-D array  Unit=N*m  AffineConversion=off
  Rotational Motion Sensor : fl_lib/Mechanical/Mechanical Sensors/Ideal Rotational Motion Sensor  reference=foundation.enum.MeasurementReference.difference  acceleration_port=false  velocity_port=true  position_port=true  wrap_angle=simscape.enum.onoff.off  offset=0 deg
  Torque Sensor : fl_lib/Mechanical/Mechanical Sensors/Ideal Torque Sensor
  R1 : PMIOPort  Side=Left
  R2 : PMIOPort  Port=2  Side=Right
  tag scope: Tq_meas=global, W=global
  wires:
  PS-Simulink Converter1/1 -> [W]
  PS-Simulink Converter2/1 -> Goto3/1
  PS-Simulink Converter3/1 -> [Tq_meas]
  connections:
  Rotational Motion Sensor/LConn1 -- Torque Sensor/RConn1 -- R2/RConn1
  Torque Sensor/RConn2 -- PS-Simulink Converter3/LConn1
  Rotational Motion Sensor/RConn2 -- PS-Simulink Converter1/LConn1
  Rotational Motion Sensor/RConn3 -- PS-Simulink Converter2/LConn1
  Mechanical Rotational Reference2/LConn1 -- Rotational Motion Sensor/RConn1
  R1/RConn1 -- Torque Sensor/LConn1

== system SMTorqueControl_PdM/Sensing Vdc ==
  PS-Simulink Converter4 : nesl_utility/PS-Simulink Converter  PhysicalDomain=network_engine_domain  SubClassName=ps_output  LeftPortType=input  RightPortType=output  PseudoPeriodic=off  Frequencies=[]  VectorFormat=1-D array  Unit=V  AffineConversion=off
  Voltage Sensor : fl_lib/Electrical/Electrical Sensors/Voltage Sensor
  + : PMIOPort  Side=Left
  - : PMIOPort  Port=2  Side=Right
  tag scope: Vdc=global
  wires:
  PS-Simulink Converter4/1 -> [Vdc]
  connections:
  Voltage Sensor/LConn1 -- +/RConn1
  Voltage Sensor/RConn2 -- -/RConn1
  PS-Simulink Converter4/LConn1 -- Voltage Sensor/RConn1

== system SMTorqueControl_PdM/Sensing iabc ==
  Current Sensor : ee_lib/Sensors & Transducers/Current Sensor (Three-Phase)  port_option=ee.enum.threePhasePort.composite
  PS-Simulink Converter : nesl_utility/PS-Simulink Converter  PhysicalDomain=network_engine_domain  SubClassName=ps_output  LeftPortType=input  RightPortType=output  PseudoPeriodic=off  Frequencies=[]  VectorFormat=1-D array  Unit=A  AffineConversion=off
  1 : PMIOPort  Side=Left
  2 : PMIOPort  Port=2  Side=Right
  tag scope: I_ABC=global
  wires:
  PS-Simulink Converter/1 -> [I_ABC]
  connections:
  1/RConn1 -- Current Sensor/LConn1
  2/RConn1 -- Current Sensor/RConn2
  Current Sensor/RConn1 -- PS-Simulink Converter/LConn1

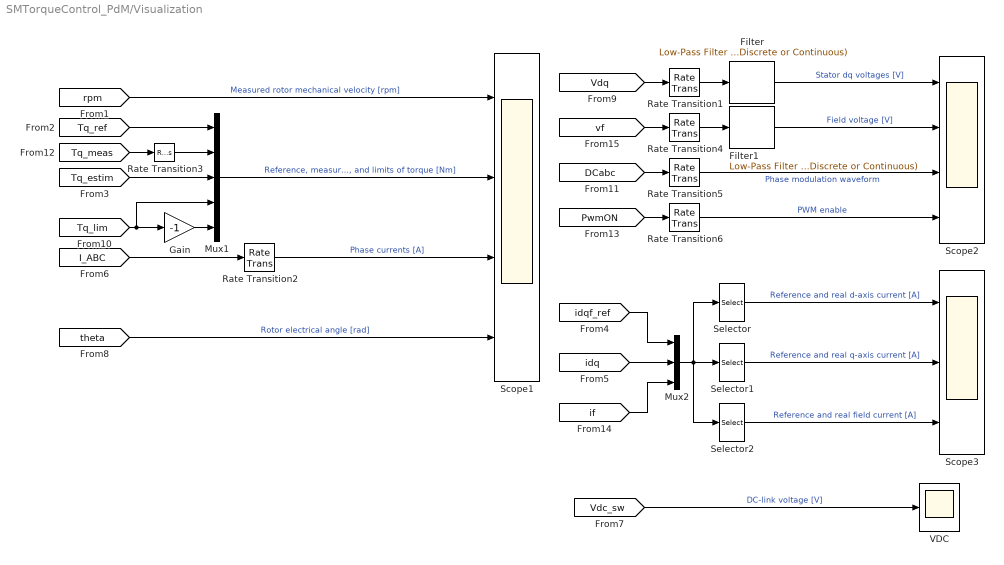
== system SMTorqueControl_PdM/Visualization ==
  Filter : eeGeneralControl/Low-Pass Filter (Discrete or Continuous)  K=1  T=0.05  B=inf  A=-inf  init_option=Inherited from block input  x0=0  Ts=Tsi
  Filter1 : eeGeneralControl/Low-Pass Filter (Discrete or Continuous)  K=1  T=0.05  B=inf  A=-inf  init_option=Inherited from block input  x0=0  Ts=Tsi
  Gain : Gain  Gain=-1
  Mux1 : Mux  Inputs=5
  Mux2 : Mux  Inputs=3
  Rate Transition{1,4..6} (4 alike) : RateTransition  OutPortSampleTime=Tsi
  Rate Transition2 : RateTransition
  Rate Transition3 : RateTransition
  Scope1 : Scope  NumInputPorts=4
      settings: ActiveDisplayYMinimum=-249.99999999999994  ActiveDisplayYMaximum=2250  DataLoggingSaveFormat=Array
  Scope2 : Scope  NumInputPorts=4
      settings: ActiveDisplayYMinimum=-110.23475  ActiveDisplayYMaximum=89.83125  DataLoggingVariableName=ScopeData3  DataLoggingSaveFormat=Array
  "Scope3 " : Scope  NumInputPorts=3
      settings: ActiveDisplayYMinimum=-147.62964  ActiveDisplayYMaximum=49.34388  DataLoggingVariableName=ScopeData2  DataLoggingSaveFormat=Array
  Selector : Selector  InputPortWidth=6  IndexOptions=Index vector (dialog)  Indices=[1 4]  OutputSizes=1
  Selector1 : Selector  InputPortWidth=6  IndexOptions=Index vector (dialog)  Indices=[2 5]  OutputSizes=1
  Selector2 : Selector  InputPortWidth=6  IndexOptions=Index vector (dialog)  Indices=[3 6]  OutputSizes=1
  VDC : Scope
      settings: ActiveDisplayYMinimum=-43.65366  ActiveDisplayYMaximum=392.90021  DataLoggingSaveFormat=Array
  wires:
  [if] -> Mux2/3
  Filter/1 -> Scope2/1  "Stator dq voltages [V]"
  [DCabc] -> Rate Transition5/1
  Rate Transition3/1 -> Mux1/2
  [Tq_ref] -> Mux1/1
  [Vdc_sw] -> VDC/1  "DC-link voltage [V]"
  [PwmON] -> Rate Transition6/1
  [rpm] -> Scope1/1  "Measured rotor mechanical velocity [rpm]"
  [Tq_meas] -> Rate Transition3/1
  Rate Transition2/1 -> Scope1/3  "Phase currents [A]"
  Mux2/1 -> Selector/1, Selector2/1, Selector1/1
  [Tq_estim] -> Mux1/3
  [idqf_ref] -> Mux2/1
  [idq] -> Mux2/2
  [Tq_lim] -> Gain/1, Mux1/4
  Filter1/1 -> Scope2/2  "Field voltage [V]"
  [theta] -> Scope1/4  "Rotor electrical angle [rad]"
  Gain/1 -> Mux1/5
  [I_ABC] -> Rate Transition2/1
  Mux1/1 -> Scope1/2  "Reference, measured, estim, and limits of torque [Nm]"
  Selector1/1 -> "Scope3 "/2  "Reference and real q-axis current [A]"
  Selector/1 -> "Scope3 "/1  "Reference and real d-axis current [A]"
  Selector2/1 -> "Scope3 "/3  "Reference and real field current [A]"
  Rate Transition4/1 -> Filter1/1
  Rate Transition1/1 -> Filter/1
  [Vdq] -> Rate Transition1/1
  [vf] -> Rate Transition4/1
  Rate Transition5/1 -> Scope2/3  "Phase modulation waveform"
  Rate Transition6/1 -> Scope2/4  "PWM enable"

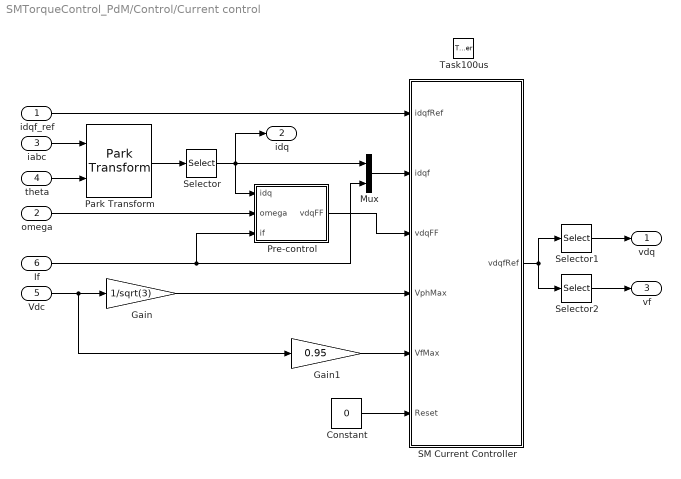
== system SMTorqueControl_PdM/Control/Current control ==
  idqf_ref : Inport
  omega : Inport  Port=2
  iabc : Inport  Port=3
  theta : Inport  Port=4
  Vdc : Inport  Port=5
  If : Inport  Port=6
  Task100us : TriggerPort  TriggerType=function-call  VariantControl=Variant  PortDimensions=1
  Constant : Constant  Value=0  SampleTime=-1
  Gain : Gain  Gain=1/sqrt(3)
  Gain1 : Gain  Gain=0.95
  Mux : Mux  Inputs=2
  Park Transform : eeTransforms/Park Transform  AxisAlignment=Q-axis  PowerInvariant=off
  Pre-control : Subsystem
  SM Current Controller : Subsystem  LoadFcn=ee_sli_rtmsupport( 'loadfcn', gcbh );  mask(SM Current Controller){Ts=-1, Tsd=Tsi, AxisPrio=Q-axis, ActZC=on, ActFF=on, Kp_id=Kp_id, Ki_id=Ki_id, Kaw_id=Kaw_id, Kp_iq=Kp_iq, Ki_iq=Ki_iq, Kaw_iq=Kaw_iq, Kp_if=Kp_if, Ki_if=Ki_if, Kaw_if=Kaw_if}
      mask prompts: Ts "physmod:ee:library:comments:control:eeSmCurrentController:SampleTime1ForInherited_MP"; Tsd "physmod:ee:library:comments:control:eeSmCurrentController:DiscretizationSampleTime_MP"; AxisPrio "physmod:ee:library:comments:control:eeSmCurrentController:AxisPrioritization_MP"; ActZC "physmod:ee:library:comments:control:eeSmCurrentController:EnableZerocancellation_MP"; ActFF "physmod:ee:library:comments:control:eeSmCurrentController:EnablePrecontrolVoltage_MP"; Kp_id "physmod:ee:library:comments:control:eeSmCurrentController:DaxisCurrentProportionalGain_MP"; Ki_id "physmod:ee:library:comments:control:eeSmCurrentController:DaxisCurrentIntegralGain_MP"; Kaw_id "physmod:ee:library:comments:control:eeSmCurrentController:DaxisCurrentAntiwindupGain_MP"; Kp_iq "physmod:ee:library:comments:control:eeSmCurrentController:QaxisCurrentProportionalGain_MP"; Ki_iq "physmod:ee:library:comments:control:eeSmCurrentController:QaxisCurrentIntegralGain_MP"; Kaw_iq "physmod:ee:library:comments:control:eeSmCurrentController:QaxisCurrentAntiwindupGain_MP"; Kp_if "physmod:ee:library:comments:control:eeSmCurrentController:FieldCurrentProportionalGain_MP"; Ki_if "physmod:ee:library:comments:control:eeSmCurrentController:FieldCurrentIntegralGain_MP"; Kaw_if "physmod:ee:library:comments:control:eeSmCurrentController:FieldCurrentAntiwindupGain_MP"
      mask help: physmod:ee:library:comments:control:eeSmCurrentController:SMCurrentController_MD
      mask init:
      | [Tsd, numZC_id, denZC_id, numZC_iq, denZC_iq, numZC_if, denZC_if] = ee.mask.initializeSmCurrentController(ActZC,Ts,Tsd,Kp_id,Ki_id,Kp_iq,Ki_iq,Kp_if,Ki_if);
      settings: CopyFcn=ee_sli_rtmsupport( 'copyfcn', gcbh );  DeleteFcn=ee_sli_rtmsupport( 'deletefcn', gcbh );  ModelCloseFcn=ee_sli_rtmsupport( 'modelclosefcn', gcbh );  PostSaveFcn=ee_sli_rtmsupport( 'postsavefcn', gcbh );  PreCopyFcn=ee_sli_rtmsupport( 'precopyfcn', gcbh );  OpenFcn=ee_sli_rtmsupport( 'openfcn', gcbh );  CloseFcn=ee_sli_rtmsupport( 'closefcn', gcbh );  PreDeleteFcn=ee_sli_rtmsupport( 'predeletefcn', gcbh );
      mask Help: web(nesl_help(gcbh))
      mask Callback Ts: ee.mask.callbackZeroCancellation(gcb);
      mask TypeOptions AxisPrio: d-q Voltage Limiter/AxisPrio
      mask Callback ActZC: ee.mask.callbackZeroCancellation(gcb);
      mask DialogControl Container2 Prompt: physmod:ee:library:comments:control:eeSmCurrentController:tab_General
      mask DialogControl Ts Prompt: Sample time (-1 for inherited)
      mask DialogControl Tsd Prompt: Discretization sample time
      mask DialogControl AxisPrio Prompt: Axis prioritization
      mask DialogControl ActZC Prompt: Enable zero-cancellation
      mask DialogControl ActFF Prompt: Enable pre-control voltage
      mask DialogControl Container3 Prompt: physmod:ee:library:comments:control:eeSmCurrentController:tab_dqControl
      mask DialogControl Kp_id Prompt: D-axis current proportional gain
      mask DialogControl Ki_id Prompt: D-axis current integral gain
      mask DialogControl Kaw_id Prompt: D-axis current anti-windup gain
      mask DialogControl Kp_iq Prompt: Q-axis current proportional gain
      mask DialogControl Ki_iq Prompt: Q-axis current integral gain
      mask DialogControl Kaw_iq Prompt: Q-axis current anti-windup gain
      mask DialogControl Container4 Prompt: physmod:ee:library:comments:control:eeSmCurrentController:tab_FieldControl
      mask DialogControl Kp_if Prompt: Field current proportional gain
      mask DialogControl Ki_if Prompt: Field current integral gain
      mask DialogControl Kaw_if Prompt: Field current anti-windup gain
  Selector : Selector  InputPortWidth=3  IndexOptions=Index vector (dialog)  Indices=[1 2]  OutputSizes=1
  Selector1 : Selector  InputPortWidth=3  IndexOptions=Index vector (dialog)  Indices=[1 2]  OutputSizes=1
  Selector2 : Selector  InputPortWidth=3  IndexOptions=Index vector (dialog)  Indices=3  OutputSizes=1
  vdq : Outport  VectorParamsAs1DForOutWhenUnconnected=off
  idq : Outport  Port=2  VectorParamsAs1DForOutWhenUnconnected=off
  vf : Outport  Port=3  VectorParamsAs1DForOutWhenUnconnected=off
  wires:
  iabc/1 -> Park Transform/1
  Park Transform/1 -> Selector/1
  theta/1 -> Park Transform/2
  idqf_ref/1 -> SM Current Controller/1(idqfRef)
  Selector/1 -> Mux/1, idq/1, Pre-control/1(idq)
  Pre-control/1(vdqFF) -> SM Current Controller/3(vdqFF)
  Vdc/1 -> Gain1/1, Gain/1
  omega/1 -> Pre-control/2(omega)
  If/1 -> Pre-control/3(if), Mux/2
  Gain/1 -> SM Current Controller/4(VphMax)
  Gain1/1 -> SM Current Controller/5(VfMax)
  Constant/1 -> SM Current Controller/6(Reset)
  SM Current Controller/1(vdqfRef) -> Selector2/1, Selector1/1
  Selector1/1 -> vdq/1
  Selector2/1 -> vf/1
  Mux/1 -> SM Current Controller/2(idqf)

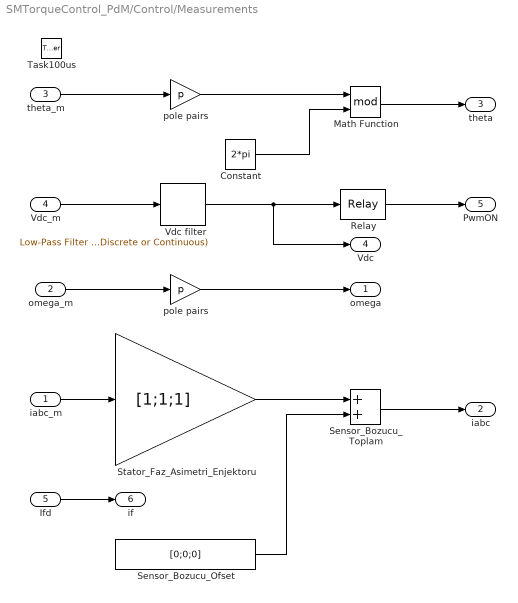
== system SMTorqueControl_PdM/Control/Measurements ==
  iabc_m : Inport
  omega_m : Inport  Port=2
  theta_m : Inport  Port=3
  Vdc_m : Inport  Port=4
  Ifd : Inport  Port=5
  Task100us : TriggerPort  TriggerType=function-call  VariantControl=Variant  PortDimensions=1
  Constant : Constant  Value=2*pi  SampleTime=-1
  Math Function : Math  Operator=mod  SignedPower=on
  Relay : Relay  OnSwitchValue=VDC_VECT(1)  OffSwitchValue=0.5*VDC_VECT(1)
  Sensor_Bozucu_Ofset : Constant  Value=[0;0;0]
  Sensor_Bozucu_Toplam : Sum
  Stator_Faz_Asimetri_Enjektoru : Gain  Gain=[1;1;1]
  Vdc filter : eeGeneralControl/Low-Pass Filter (Discrete or Continuous)  K=1  T=0.005  B=inf  A=-inf  init_option=Inherited from block input  x0=0  Ts=-1
  pole pairs : Gain  Gain=p
  "pole pairs " : Gain  Gain=p
  omega : Outport  VectorParamsAs1DForOutWhenUnconnected=off
  iabc : Outport  Port=2  VectorParamsAs1DForOutWhenUnconnected=off
  theta : Outport  Port=3  VectorParamsAs1DForOutWhenUnconnected=off
  Vdc : Outport  Port=4  VectorParamsAs1DForOutWhenUnconnected=off
  PwmON : Outport  Port=5  VectorParamsAs1DForOutWhenUnconnected=off
  if : Outport  Port=6  VectorParamsAs1DForOutWhenUnconnected=off
  wires:
  Constant/1 -> Math Function/2
  Sensor_Bozucu_Toplam/1 -> iabc/1
  iabc_m/1 -> Stator_Faz_Asimetri_Enjektoru/1
  Ifd/1 -> if/1
  Relay/1 -> PwmON/1
  omega_m/1 -> pole pairs/1
  Math Function/1 -> theta/1
  Vdc_m/1 -> Vdc filter/1
  Sensor_Bozucu_Ofset/1 -> Sensor_Bozucu_Toplam/2
  theta_m/1 -> "pole pairs "/1
  Vdc filter/1 -> Vdc/1, Relay/1
  "pole pairs "/1 -> Math Function/1
  pole pairs/1 -> omega/1
  Stator_Faz_Asimetri_Enjektoru/1 -> Sensor_Bozucu_Toplam/1
